simulink model "Stabilizer_QDrone_QGC_OF_RYPI_FA"  (Simulink 9.3)
settings: Solver=ode2  StartTime=0.0  StopTime=inf  FixedStep=0.001  RelTol=1e-3  EnableMultiTasking=on
InitFcn:
  | addpath(fileparts(get_param(bdroot,'FileName')));setup_project;
values from neighbouring files (symbols this model uses):
  x = xp + K*(z-xp(1))    [qdrone_baro_height_kalman.m]    (also in qdrone_baro_height_kalman_smooth.m)
undefined symbols (not defined in the file or in its folder): datetime, FlowAssist_, gcbh, HIL, HILTiming_, m, OpticalFlow_, qc_get_step_size, QDrone_, RollYawPI_, saved_data, Stabilizer_, TimingDiagnostics_NoVideo_Repeat_, video_display_show
undefined symbols (not defined in the file): JPEG
libraries: quarc_library x40, simulink_extras x5, simulink x4
(part 2 of 2)

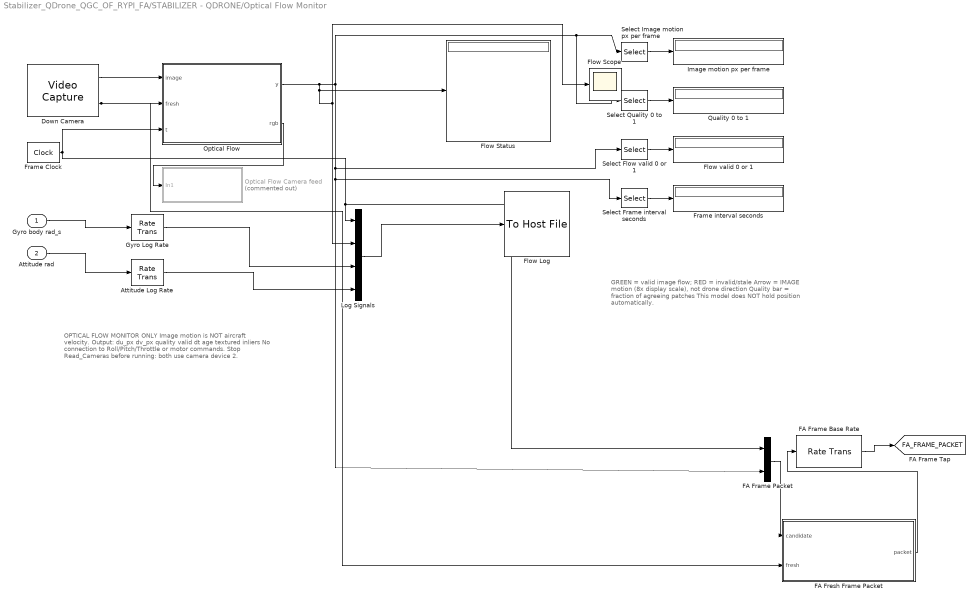
== system Stabilizer_QDrone_QGC_OF_RYPI_FA/STABILIZER - QDRONE/Optical Flow Monitor ==
  note: GREEN = valid image flow; RED = invalid/stale
      | Arrow = IMAGE motion (8x display scale), not drone direction
      | Quality bar = fraction of agreeing patches
      | This model does NOT hold position automatically.
  note: OPTICAL FLOW MONITOR ONLY
      | Image motion is NOT aircraft velocity.
      | Output: du_px dv_px quality valid dt age textured inliers
      | No connection to Roll/Pitch/Throttle or motor commands.
      | Stop Read_Cameras before running: both use camera device 2.
  Gyro body rad_s : Inport
  Attitude rad : Inport  Port=2
  Attitude Log Rate : RateTransition  OutPortSampleTime=0.033
  Down Camera : quarc_library/Multimedia/Video Capture  source=device  device=2  filename=sample_movie.mov  value=[0 0; 0 0]  resolution=640 x 480  width=640  height=480  output_format=MATLAB greyscale (HxW)  data_type=uint8  sample_time=0.033  brightness_override=off  brightness=50.0  contrast_override=off  contrast=50.0  hue_override=off  hue=50.0  saturation_override=off  saturation=50.0  sharpness_override=off  sharpness=50.0  gamma_override=off  gamma=50.0  coloreffect_override=off  coloreffect=None  whitebalance_override=off  whitebalance=50.0  backlightcompensation_override=off  backlightcompensation=0.0  gain_override=off  gain=50.0  pan_override=off  pan=50.0  tilt_override=off  tilt=50.0  roll_override=off  roll=50.0  zoom_override=off  zoom=0.0  exposure_override=off  exposure=50.0  iris_override=off  iris=50.0  focus_override=off  focus=0.0
      settings: SourceProductName=QUARC Targets
  FA Frame Base Rate : RateTransition  OutPortSampleTime=0.001
  FA Frame Packet : Mux  Inputs=2
  FA Fresh Frame Packet : MATLAB Function  TreatAsAtomicUnit=on
  Flow Log : quarc_library/Sinks/To Host/To Host File  file_name=saved_data/%m/OpticalFlow_%{char(datetime)}.mat  variable_name=optical_flow_data  decimation=1  sample_time=0.033  file_format=MAT-file v.5  options=No header or footer  append=off  final_file_name=saved_data/Stabilizer_QDrone_QGC_OF_RYPI_FA/OpticalFlow_10-Nov-2026 20-24-47.mat  bitrate=2000000
      settings: SourceProductName=The database C:\Users\user\AppData\Roaming\MathWorks\MATLAB\R2017a\slblocks_master.db is locked, or a table in the database is locked. (database is locked)
  Flow Scope : Scope
  Flow Status : Display
  Flow valid 0 or 1 : Display
  Frame Clock : DigitalClock  SampleTime=0.033
  Frame interval seconds : Display
  Gyro Log Rate : RateTransition  OutPortSampleTime=0.033
  Image motion px per frame : Display
  Log Signals : Mux
  Optical Flow : MATLAB Function  TreatAsAtomicUnit=on
  Optical Flow Camera feed : Subsystem  Commented=on  LoadFcn=set_param(gcbh, 'UserData', gcb);  StartFcn=video_display_show([gcb, '/Video Display'], 'add', gcb);  mask(Video Compressed Display){algorithm=JPEG, quality=50, sample_time=-1, use_hardware=on}
      mask prompts: algorithm "Compression algorithm:"; quality "Compression quality (0-100):"; sample_time "Sample time (seconds):"; use_hardware "Use hardware acceleration for video display"
      mask help: Displays a video stream on the host, using compression to minimize bandwidth.
      mask init:
      | qc_set_display('Video\nCompressed\nDisplay');
      settings: UndoDeleteFcn=set_param(gcbh, 'UserData', gcb);  OpenFcn=video_display_show([gcb, '/Video Display'], 'show', gcb);  PreDeleteFcn=video_display_show([gcb, '/Video Display'], 'delete');
      settings: CopyFcn=|
      | set_param(gcbh, 'UserData', gcb);
      | set_param(gcbh, 'LinkStatus', 'none');
      settings: NameChangeFcn=|
      | video_display_show([get_param(gcbh, 'UserData'), '/Video Display'], 'rename', [gcb, '/Video Display']);
      | video_display_show([gcb, '/Video Display'], 'add', gcb);
      | set_param(gcbh, 'UserData', gcb);
      mask Help: web(qc_get_block_help_path(gcb));
      mask TypeOptions algorithm: Image Compress/algorithm
      mask TypeOptions quality: Image Compress/quality
      mask TypeOptions sample_time: Video Display/sample_time
      mask TypeOptions use_hardware: Video Display/use_hardware
      mask Display:
      | patch([0.98591 0.98591 0.62618 0.59072 0.56147   0.536   0.536  0.5441 0.56912 0.59207 0.60881 0.62276 0.63527 0.64364  0.6485  0.6485 0.64706 0.64499 0.63662 0.62411 0.61232 0.59837 0.58307 0.56147   0.536   0.536  0.5441  0.5747 0.60953 0.63662 0.67001  0.7034 0.72851 0.75425 0.77927 0.80294 0.82454 0.84119 0.85865 0.87395 0.88574 0.89339  0.8969 0.89969 0.89969 0.89267  0.8816 0.87044 0.85649  0.8384 0.81824 0.80294 0.78764 0.77513 0.76676 0.75776 0.76397 0.77513 0.79178 0.80987 0.82796 0.84326 0.86207 0.98528],[0.18689 0.05522 0.05522 0.05171 0.05171    0.05 0.18338 0.18338 0.19148 0.20435 0.22298 0.24863 0.28589 0.33125 0.38138 0.55139 0.59801 0.63761 0.68189 0.72149 0.74939 0.76694 0.77855 0.79367 0.79952 0.92768 0.92768 0.92768 0.92417 0.92066 0.91364  0.9032 0.89384 0.88106 0.86594 0.85073 0.82634 0.80537 0.77855 0.74363 0.70403 0.65858 0.61079 0.59099 0.41513 0.37202 0.31847 0.29048 0.25556 0.23342  0.2102 0.19382 0.18221 0.17285 0.16943 0.16124  0.1589 0.16241 0.16709 0.17168  0.1787 0.18221 0.18689 0.18689],[0.9,0.90,0.91])
      | patch([0.536 0.52601 0.46823 0.44528 0.41603 0.39101 0.35555 0.33116 0.31451 0.29291  0.2804 0.26717 0.25322 0.23999 0.22406 0.20732 0.19337 0.17528 0.15935 0.14396 0.13217 0.11759 0.10922 0.10085 0.09671 0.09392 0.09041 0.08906 0.08906 0.09464  0.0995 0.10778 0.11894 0.13145 0.14675 0.16349 0.17672 0.19409 0.20732 0.22406 0.23999 0.26159 0.27833 0.29849 0.31793 0.33602 0.35411 0.37085 0.39245 0.41603   0.536   0.536 0.53159 0.46409   0.446 0.42026 0.39587 0.37571 0.36113 0.34925 0.34088 0.33809 0.33809 0.34088 0.34583 0.35627 0.36392 0.38129 0.39587 0.41117 0.42719 0.44672  0.4676 0.48353 0.48353 0.52394   0.536],[0.05 0.04829 0.04712 0.04712 0.04829 0.05063 0.05405 0.05873 0.06107 0.06692 0.07043 0.07619 0.08087 0.08672 0.09482 0.10652 0.11696 0.13325  0.1508 0.17168 0.19499 0.22415 0.25439 0.28472 0.31379 0.35456 0.38489 0.41513 0.58055 0.63878 0.68774 0.72149 0.75641 0.78089 0.80537 0.82859 0.84029 0.85658 0.86594 0.87404  0.8834 0.89267 0.90086 0.90788 0.91247 0.91832 0.92066   0.923 0.92651 0.92768 0.92768 0.79952 0.79952 0.79952 0.79718 0.78899 0.77153 0.75056 0.72149 0.68072 0.62249  0.5549 0.41396 0.37085 0.33242 0.28121 0.25205 0.22181 0.20552 0.19499 0.18572 0.18221 0.17753 0.17636 0.17753  0.1787  0.1787],[0.9,0.90,0.91])
      | disp('Video\nCompressed\nDisplay');
  Quality 0 to 1 : Display
  Select Flow valid 0 or 1 : Selector  InputPortWidth=8  IndexOptions=Index vector (dialog)  Indices=4  OutputSizes=1
  Select Frame interval seconds : Selector  InputPortWidth=8  IndexOptions=Index vector (dialog)  Indices=5  OutputSizes=1
  Select Image motion px per frame : Selector  InputPortWidth=8  IndexOptions=Index vector (dialog)  Indices=[1 2]  OutputSizes=1
  Select Quality 0 to 1 : Selector  InputPortWidth=8  IndexOptions=Index vector (dialog)  Indices=3  OutputSizes=1
  tag scope: FA_FRAME_PACKET=global
  wires:
  Select Frame interval seconds/1 -> Frame interval seconds/1
  Select Flow valid 0 or 1/1 -> Flow valid 0 or 1/1
  Select Quality 0 to 1/1 -> Quality 0 to 1/1
  Select Image motion px per frame/1 -> Image motion px per frame/1
  Optical Flow/2(rgb) -> Optical Flow Camera feed/1(In1)
  Attitude Log Rate/1 -> Log Signals/4
  Gyro Log Rate/1 -> Log Signals/3
  Log Signals/1 -> Flow Log/1
  Attitude rad/1 -> Attitude Log Rate/1
  Gyro body rad_s/1 -> Gyro Log Rate/1
  Optical Flow/1(y) -> FA Frame Packet/2, Select Frame interval seconds/1, Select Flow valid 0 or 1/1, Select Quality 0 to 1/1, Select Image motion px per frame/1, Log Signals/2, Flow Scope/1, Flow Status/1
  Frame Clock/1 -> Log Signals/1, FA Frame Packet/1, Optical Flow/3(t)
  Down Camera/2 -> Optical Flow/2(fresh), FA Fresh Frame Packet/2(fresh)
  Down Camera/1 -> Optical Flow/1(image)
  FA Frame Packet/1 -> FA Fresh Frame Packet/1(candidate)
  FA Frame Base Rate/1 -> [FA_FRAME_PACKET]
  FA Fresh Frame Packet/1(packet) -> FA Frame Base Rate/1

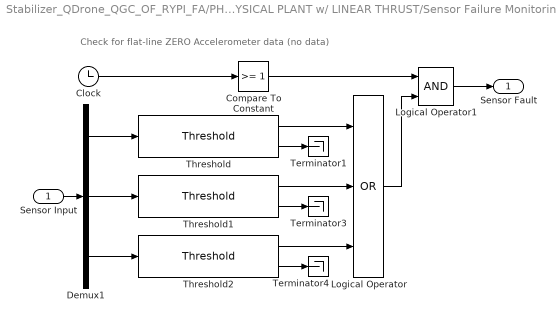
== system Stabilizer_QDrone_QGC_OF_RYPI_FA/PHYSICAL PLANT w/ LINEAR THRUST/Sensor Failure Monitoring/Sensor Failure (Accelerometer) ==
  note: Check for flat-line ZERO Accelerometer data (no data)
  Sensor Input : Inport
  Clock : Clock
  Compare To Constant : simulink/Logic and Bit Operations/Compare To Constant  relop=>=  const=1  OutDataTypeStr=boolean
  Demux1 : Demux  Outputs=3
  Logical Operator : Logic  Operator=OR  Inputs=3  AllPortsSameDT=off  OutDataTypeStr=boolean
  Logical Operator1 : Logic  AllPortsSameDT=off  OutDataTypeStr=boolean
  Terminator1 : Terminator
  Terminator3 : Terminator
  Terminator4 : Terminator
  Threshold : quarc_library/Discontinuities/Threshold  operator===  param_src=Specify via dialog  threshold=0  duration=1
      settings: SourceProductName=The database C:\Users\user\AppData\Roaming\MathWorks\MATLAB\R2017a\slblocks_master.db is locked, or a table in the database is locked. (database is locked)
  Threshold1 : quarc_library/Discontinuities/Threshold  operator===  param_src=Specify via dialog  threshold=0  duration=1
      settings: SourceProductName=The database C:\Users\user\AppData\Roaming\MathWorks\MATLAB\R2017a\slblocks_master.db is locked, or a table in the database is locked. (database is locked)
  Threshold2 : quarc_library/Discontinuities/Threshold  operator===  param_src=Specify via dialog  threshold=0  duration=1
      settings: SourceProductName=The database C:\Users\user\AppData\Roaming\MathWorks\MATLAB\R2017a\slblocks_master.db is locked, or a table in the database is locked. (database is locked)
  Sensor Fault : Outport
  wires:
  Clock/1 -> Compare To Constant/1
  Threshold/1 -> Logical Operator/1
  Threshold1/1 -> Logical Operator/2
  Compare To Constant/1 -> Logical Operator1/1
  Logical Operator1/1 -> Sensor Fault/1
  Sensor Input/1 -> Demux1/1
  Threshold2/2 -> Terminator4/1
  Threshold2/1 -> Logical Operator/3
  Demux1/1 -> Threshold/1
  Demux1/3 -> Threshold2/1
  Demux1/2 -> Threshold1/1
  Logical Operator/1 -> Logical Operator1/2
  Threshold1/2 -> Terminator3/1
  Threshold/2 -> Terminator1/1

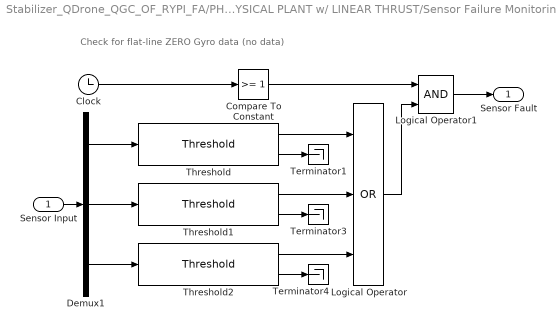
== system Stabilizer_QDrone_QGC_OF_RYPI_FA/PHYSICAL PLANT w/ LINEAR THRUST/Sensor Failure Monitoring/Sensor Failure (Gyroscope) ==
  note: Check for flat-line ZERO Gyro data (no data)
  Sensor Input : Inport
  Clock : Clock
  Compare To Constant : simulink/Logic and Bit Operations/Compare To Constant  relop=>=  const=1  OutDataTypeStr=boolean
  Demux1 : Demux  Outputs=3
  Logical Operator : Logic  Operator=OR  Inputs=3  AllPortsSameDT=off  OutDataTypeStr=boolean
  Logical Operator1 : Logic  AllPortsSameDT=off  OutDataTypeStr=boolean
  Terminator1 : Terminator
  Terminator3 : Terminator
  Terminator4 : Terminator
  Threshold : quarc_library/Discontinuities/Threshold  operator===  param_src=Specify via dialog  threshold=0  duration=1
      settings: SourceProductName=The database C:\Users\user\AppData\Roaming\MathWorks\MATLAB\R2017a\slblocks_master.db is locked, or a table in the database is locked. (database is locked)
  Threshold1 : quarc_library/Discontinuities/Threshold  operator===  param_src=Specify via dialog  threshold=0  duration=1
      settings: SourceProductName=The database C:\Users\user\AppData\Roaming\MathWorks\MATLAB\R2017a\slblocks_master.db is locked, or a table in the database is locked. (database is locked)
  Threshold2 : quarc_library/Discontinuities/Threshold  operator===  param_src=Specify via dialog  threshold=0  duration=1
      settings: SourceProductName=The database C:\Users\user\AppData\Roaming\MathWorks\MATLAB\R2017a\slblocks_master.db is locked, or a table in the database is locked. (database is locked)
  Sensor Fault : Outport
  wires:
  Threshold/2 -> Terminator1/1
  Threshold1/2 -> Terminator3/1
  Logical Operator/1 -> Logical Operator1/2
  Demux1/2 -> Threshold1/1
  Demux1/3 -> Threshold2/1
  Demux1/1 -> Threshold/1
  Threshold2/1 -> Logical Operator/3
  Threshold2/2 -> Terminator4/1
  Sensor Input/1 -> Demux1/1
  Logical Operator1/1 -> Sensor Fault/1
  Compare To Constant/1 -> Logical Operator1/1
  Threshold1/1 -> Logical Operator/2
  Threshold/1 -> Logical Operator/1
  Clock/1 -> Compare To Constant/1

== system Stabilizer_QDrone_QGC_OF_RYPI_FA/STABILIZER - QDRONE/Optical Flow Monitor/Optical Flow Camera feed ==
  In1 : Inport
  Channel : quarc_library/Signal Routing/Channel  channel=0  buffer_size=1
  Image Compress : quarc_library/Image Processing/Generic/Image Compress  algorithm=JPEG  source=Internal dialog parameter  quality=quality  output_dim=-1
  Video Display : quarc_library/Multimedia/Video Display  Tag=Stabilizer_QDrone_QGC_OF_RYPI_FA/STABILIZER - QDRONE/Optical Flow Monitor/Optical Flow Camera feed/Video Display  sample_time=sample_time  use_hardware=on
  wires:
  Channel/1 -> Video Display/1
  In1/1 -> Image Compress/1
  Image Compress/1 -> Channel/1

== matlab function PHYSICAL PLANT w// LINEAR THRUST/roll and pitch approximation from accelerometer ==
  data: roll_acc output double; pitch_acc output double; acc_body input double
function [roll_acc, pitch_acc]   = fcn(acc_body)
%#eml
n = norm(acc_body,2);
if n>eps
    acc_body = acc_body/n; 
else
    acc_body = [0 0 1]';
end

roll_acc = atan2(acc_body(2),acc_body(3));
pitch_acc = atan2( -acc_body(1), acc_body(2)*sin(roll_acc)+acc_body(3)*cos(roll_acc));

== matlab function STABILIZER - QDRONE/Optical Flow Monitor/Optical Flow ==
  data: image input double; y output double; fresh input double; t input double; rgb output double
function [y,rgb]=run(image,fresh,t)
%#codegen
y=qdrone_of_step(image,fresh,t,false);
rgb=qdrone_of_overlay(image,y);
end

== matlab function Communication/Detect Communication loss/MATLAB Function ==
  settings: updateMethod=DISCRETE
  data: time input double; stream_connection_loss output double; state input double; error input double; ms_time input double; data_loss output double
function [stream_connection_loss , data_loss] = fcn(time, state, error, ms_time)
% signals(1) = throttle
% signals(2) = arm

persistent ms_time_prev
    if isempty(ms_time_prev)
        ms_time_prev = 0;
    end

stream_connection_loss = 0;
data_loss = 0;
if time > 3
    if ((state ~= 2)&&(error < 0))
        % stream connection is not established correctly
        stream_connection_loss = 1;
    end

    if (ms_time == ms_time_prev)
        % data is stale
        data_loss = 1;
    end
end

ms_time_prev = ms_time;

== matlab function STABILIZER - QDRONE/RYPI Allocator Feedback ==
  settings: updateMethod=DISCRETE  sampleTime=0.001
  data: motor input double size=[4 1]; residual output double size=[3 1]; rawTorque input double size=[3 1]; limitedTorque input double size=[3 1]; inverseMixer input double size=[4 4]
function residual=feedback(motor,rawTorque,limitedTorque,inverseMixer)
%#codegen
residual=qdrone_ry_aw_step(motor,rawTorque,limitedTorque,inverseMixer);
end

== matlab function STABILIZER - QDRONE/Yaw Integral Controller ==
  settings: updateMethod=DISCRETE  sampleTime=0.001
  data: errorRate input double size=[3 1]; term output double size=[3 1]; angles input double size=[3 1]; gyro input double size=[3 1]; residual input double size=[3 1]; arm input double; throttle input double; mode input double; enable input double size=[2 1]; config input double size=[8 1]; reset input double; diagnostic output double size=[10 1]
function [term,diagnostic]=step(errorRate,angles,gyro,residual,arm,throttle,mode,enable,config,reset)
%#codegen
[term,diagnostic]=qdrone_ry_pi_step(errorRate,angles,gyro,residual,arm,throttle,mode,enable,config,reset);
end

== matlab function STABILIZER - QDRONE/FA Mode Decoder ==
  settings: updateMethod=DISCRETE  sampleTime=0.001
  data: raw input double size=1; base output double size=1; request output double size=1
function [base,request]=decode(raw)
%#codegen
base=double(raw==1);request=double(raw==2);
end

== matlab function STABILIZER - QDRONE/Flow Assist ==
  settings: updateMethod=DISCRETE  sampleTime=0.001
  data: command input double size=[3 1]; out output double size=[3 1]; flow input double size=[8 1]; frameTime input double size=1; gyro input double size=[3 1]; attitude input double size=[3 1]; arm input double size=1; throttle input double size=1; mode input double size=1; request input double size=1; config input double size=[13 1]; rotation input double size=[3 3]; time input double size=1; diagnostic output double size=[16 1]
function [out,diagnostic]=assist(command,flow,frameTime,gyro,attitude,arm,throttle,mode,request,config,rotation,time)
%#codegen
[out,diagnostic]=qdrone_fa_step(command,flow,frameTime,gyro,attitude,arm,throttle,mode,request,config,rotation,time);
end

== matlab function STABILIZER - QDRONE/Optical Flow Monitor/FA Fresh Frame Packet ==
  settings: updateMethod=DISCRETE  sampleTime=0.033
  data: candidate input double size=[9 1]; packet output double size=[9 1]; fresh input double size=1
function packet=holdFrame(candidate,fresh)
%#codegen
persistent held
if isempty(held),held=zeros(9,1);end
if candidate(1)<held(1),held=zeros(9,1);end
if fresh,held=candidate;end
packet=held;
end

== matlab function PHYSICAL PLANT w// LINEAR THRUST/Red - Low Voltage Green - Armed Blue - Disarmed/MATLAB Function LED Color Assignment ==
  data: arm input double; value output double; low_battery input double
function value = fcn(arm, low_battery)

if low_battery
    value = 1;
elseif arm
    value = 2;
else 
    value = 3;
end
